simulink model "imu_filters"  (R2026b)
settings: Solver=FixedStepDiscrete  FixedStep=dt
undefined symbols (not defined in the file or in its folder): alpha, DiscIntNeverNeededParam, dt, K
settings Model: Creator=Max  LastModifiedBy=Max

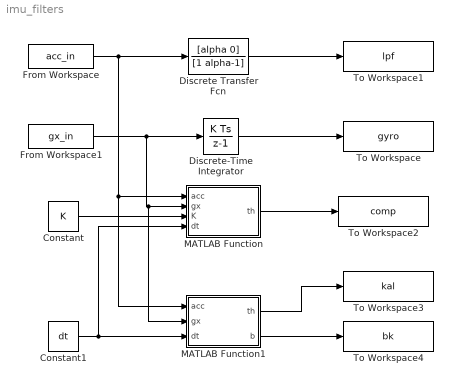
== system imu_filters ==
  Constant : Constant  Value=K
  Constant1 : Constant  Value=dt
  Discrete Transfer Fcn : DiscreteTransferFcn  Numerator=[alpha 0]  Denominator=[1 alpha-1]  InitialStates=dt
  Discrete-Time Integrator : DiscreteIntegrator  SampleTime=dt  ICPrevOutput=DiscIntNeverNeededParam  ICPrevScaledInput=DiscIntNeverNeededParam
  From Workspace : FromWorkspace  VariableName=acc_in  SampleTime=dt  Interpolate=off  OutputAfterFinalValue=Holding final value
  From Workspace1 : FromWorkspace  VariableName=gx_in  SampleTime=dt  Interpolate=off  OutputAfterFinalValue=Holding final value
  MATLAB Function : MATLAB Function  TreatAsAtomicUnit=on
  MATLAB Function1 : MATLAB Function  TreatAsAtomicUnit=on
  To Workspace : ToWorkspace  VariableName=gyro  SampleTime=-1
  To Workspace1 : ToWorkspace  VariableName=lpf  SampleTime=-1
  To Workspace2 : ToWorkspace  VariableName=comp  SampleTime=-1
  To Workspace3 : ToWorkspace  VariableName=kal  SampleTime=-1
  To Workspace4 : ToWorkspace  VariableName=bk  SampleTime=-1
  wires:
  From Workspace/1 -> MATLAB Function1/1(acc), MATLAB Function/1(acc), Discrete Transfer Fcn/1
  Discrete Transfer Fcn/1 -> To Workspace1/1
  Discrete-Time Integrator/1 -> To Workspace/1
  MATLAB Function/1(th) -> To Workspace2/1
  From Workspace1/1 -> MATLAB Function1/2(gx), MATLAB Function/2(gx), Discrete-Time Integrator/1
  Constant/1 -> MATLAB Function/3(K)
  Constant1/1 -> MATLAB Function/4(dt), MATLAB Function1/3(dt)
  MATLAB Function1/1(th) -> To Workspace3/1
  MATLAB Function1/2(b) -> To Workspace4/1

== matlab function imu_filters/MATLAB Function1 ==
  data: acc input; th output; gx input; dt input; b output
function [th, b] = fcn(acc, gx, dt)
[th, b] = kalman_filter(acc, gx, dt);

== matlab function imu_filters/MATLAB Function ==
  data: acc input; th output; gx input; K input; dt input
function th = fcn(acc, gx, K, dt)
th = complementary_filter(acc, gx, K, dt);
